simulink model "sens_odom_compute"  (R2026b)
settings: Solver=VariableStepAuto
values from neighbouring files (symbols this model uses):
  D = zeros(nx, ny, 'uint8')    [sens_lidar2d_fast.m]
  P = (P + P.')/2    [sens_nav_ekf.m]
undefined symbols (not defined in the file or in its folder): Ts
libraries: simulink x1
settings Model: Creator=aomar  LastModifiedBy=aomar

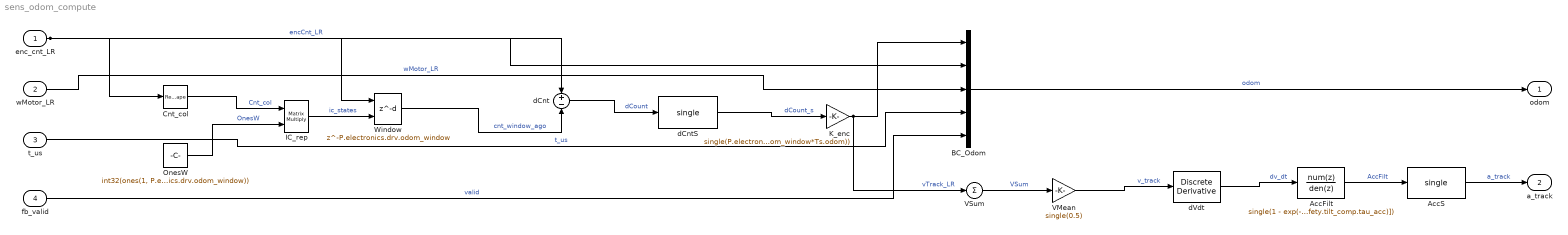
== system sens_odom_compute ==
  enc_cnt_LR : Inport  OutDataTypeStr=int32  PortDimensions=2  SampleTime=Ts.ctrl
  wMotor_LR : Inport  Port=2  OutDataTypeStr=single  PortDimensions=2  SampleTime=Ts.ctrl
  t_us : Inport  Port=3  OutDataTypeStr=uint32  PortDimensions=1  SampleTime=Ts.ctrl
  fb_valid : Inport  Port=4  OutDataTypeStr=boolean  PortDimensions=1  SampleTime=Ts.ctrl
  AccFilt : DiscreteTransferFcn  Numerator=single(1 - exp(-Ts.odom/P.electronics.safety.tilt_comp.tau_acc))  Denominator=single([1 -exp(-Ts.odom/P.electronics.safety.tilt_comp.tau_acc)])  SampleTime=Ts.ctrl
  AccS : DataTypeConversion  OutDataTypeStr=single  RndMeth=Nearest  SaturateOnIntegerOverflow=off
  BC_Odom : BusCreator  Inputs=5  OutDataTypeStr=Bus: Bus_OdomMeas  NonVirtualBus=on
      settings: InheritFromInputs=off
  Cnt_col : Reshape  OutputDimensionality=Column vector (2-D)
  IC_rep : Product  Multiplication=Matrix(*)  OutDataTypeStr=int32
  K_enc : Gain  Gain=single(P.electronics.drv.K_enc/(P.electronics.drv.odom_window*Ts.odom))  OutDataTypeStr=Inherit: Same as input  ParamDataTypeStr=Inherit: Same as input
  OnesW : Constant  Value=int32(ones(1, P.electronics.drv.odom_window))  VectorParams1D=off  OutDataTypeStr=int32
  VMean : Gain  Gain=single(0.5)  ParamDataTypeStr=Inherit: Same as input
  VSum : Sum  Inputs=+
  Window : Delay  DelayLength=P.electronics.drv.odom_window  InitialConditionSource=Input port  SampleTime=Ts.ctrl
      settings: InputPortMap=u0,p4
  dCnt : Sum  Inputs=+-  OutDataTypeStr=int32
  dCntS : DataTypeConversion  OutDataTypeStr=single  ConvertRealWorld=Stored Integer (SI)  SaturateOnIntegerOverflow=off  RndMeth=Floor
  dVdt : simulink/Discrete/Discrete Derivative  gainval=1  ICPrevScaledInput=0  OutMin=[]  OutMax=[]  OutDataType=fixdt(1, 16)  OutScaling=2^-10  DoSatur=off
  odom : Outport  OutDataTypeStr=Bus: Bus_OdomMeas
  a_track : Outport  Port=2  OutDataTypeStr=single
  wires:
  enc_cnt_LR/1 -> Window/1, Cnt_col/1, dCnt/1, BC_Odom/2  "encCnt_LR"
  wMotor_LR/1 -> BC_Odom/3  "wMotor_LR"
  t_us/1 -> BC_Odom/4  "t_us"
  fb_valid/1 -> BC_Odom/5  "valid"
  Cnt_col/1 -> IC_rep/1  "Cnt_col"
  OnesW/1 -> IC_rep/2  "OnesW"
  IC_rep/1 -> Window/2  "ic_states"
  Window/1 -> dCnt/2  "cnt_window_ago"
  dCnt/1 -> dCntS/1  "dCount"
  dCntS/1 -> K_enc/1  "dCount_s"
  K_enc/1 -> BC_Odom/1, VSum/1  "vTrack_LR"
  BC_Odom/1 -> odom/1  "odom"
  VSum/1 -> VMean/1  "VSum"
  VMean/1 -> dVdt/1  "v_track"
  dVdt/1 -> AccFilt/1  "dv_dt"
  AccFilt/1 -> AccS/1  "AccFilt"
  AccS/1 -> a_track/1  "a_track"
